simulink model "tutorial02_math"  (R2025a)
settings: Solver=VariableStepAuto  StartTime=0.0  StopTime=10.0  RelTol=1e-3
settings Model: Creator=xing2  LastModifiedBy=xing2

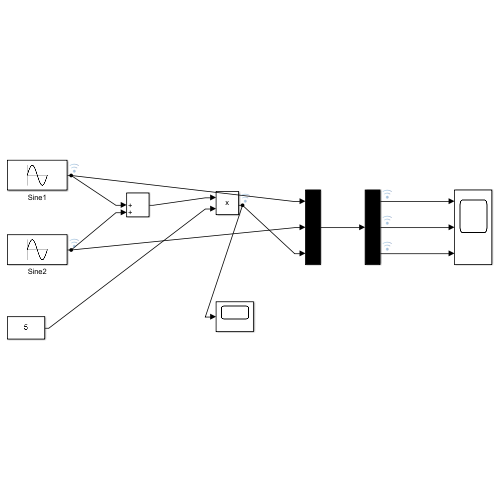
[thumbnail: Simulink's stored preview of the top-level diagram]
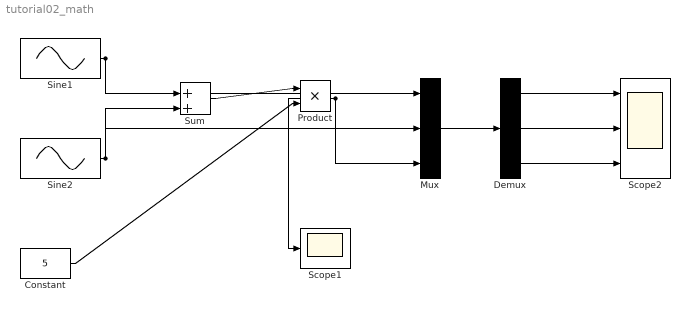
== system tutorial02_math ==
  Constant : Constant  Value=5
  Demux : Demux  Outputs=3
  Mux : Mux  Inputs=3
  Product : Product
  Scope1 : Scope
  Scope2 : Scope  NumInputPorts=3
  Sine1 : Sin  SampleTime=0
  Sine2 : Sin  Frequency=3  SampleTime=0
  Sum : Sum  Inputs=|++
  wires:
  Sine1/1 -> Sum/1, Mux/1
  Sine2/1 -> Sum/2, Mux/2
  Sum/1 -> Product/1
  Constant/1 -> Product/2
  Product/1 -> Scope1/1, Mux/3
  Mux/1 -> Demux/1
  Demux/1 -> Scope2/1
  Demux/2 -> Scope2/2
  Demux/3 -> Scope2/3
